simulink model "ZT_VehCtrl_18B_CAN"  (R2018b)
settings: Solver=FixedStepAuto  StartTime=0.0  StopTime=inf  FixedStep=0.005  RelTol=1e-3
InitFcn:
  | mbd_mpc_consistency_checks(bdroot(gcs));
values from neighbouring files (symbols this model uses):
  BatoverTempTh = single(80)    [VCU_INIT.m]
  BRS_PwrValid = single(5)    [VCU_INIT.m]
  BRSEnSpdTh1 = single(10)    [VCU_INIT.m]
  BRSEnSpdTh2 = single(20)    [VCU_INIT.m]
  MCUTempAlarmTh = single (60)    [VCU_INIT.m]
  mps2kmh = single(3.6)    [VCU_INIT.m]
  MtrPwrFac = single(1/9550)    [VCU_INIT.m]
  MtrTempAlarmTh = single (50)    [VCU_INIT.m]
  Padle1Signal1_Th = [PadleSignal1_min,PadleSignal1_max]    [VCU_INIT.m]
  Padle1Signal2_Th = [PadleSignal2_min,PadleSignal2_max]    [VCU_INIT.m]
  PadleSignal1_max = 3.84    [VCU_INIT.m]
  PadleSignal1_min = 0.75    [VCU_INIT.m]
  PadleSignal2_max = 1.92    [VCU_INIT.m]
  PadleSignal2_min = 0.375    [VCU_INIT.m]
  PadleValid = 0.05    [VCU_INIT.m]
  PwrLimFactor = single(0.5)    [VCU_INIT.m]
  Ratio = single(1)    [VCU_INIT.m]
  rpm2mps = single(2*pi/60 * WhlRadius/Ratio)    [VCU_INIT.m]
  SOCLowTh = single(20)    [VCU_INIT.m]
  VehPwrBackwardMax = VehPwrMax * single(0.3)    [VCU_INIT.m]
  VehPwrMax = single(MtrPwrMax * 4)    [VCU_INIT.m]
  VehTrqBackwardMax = VehTrqMax * single(0.3)    [VCU_INIT.m]
  VehTrqMax = single(MtrTrqMax * Ratio *4)    [VCU_INIT.m]
  WhlRadius = single(1)    [VCU_INIT.m]
undefined symbols (not defined in the file or in its folder): Delay_Charge, Delay_Discharge, fifo_0_vect, fifo_1_vect, LQFP, pts1_fifo_0_vect, pts1_fifo_1_vect, pts2_fifo_0_vect, pts2_fifo_1_vect, pts3_fifo_0_vect, pts3_fifo_1_vect, pts4_fifo_0_vect, pts4_fifo_1_vect
libraries: mbd_mpc574x_ec_toolbox x157, canmsglib x74, simulink x38
(part 8 of 12)

== system ZT_VehCtrl_18B_CAN/SigIn/CAN0 /BMS Statistic_Cell ExtremumIndex Infor/UNPACK ==
  ID : Inport
  data : Inport  Port=2
  length : Inport  Port=3
  timestamp : Inport  Port=4
  Action Port : ActionPort
  Bus Creator : BusCreator  Inputs=7  OutDataTypeStr=Bus: CAN_MESSAGE_BUS  NonVirtualBus=on
  Bus Creator1 : BusCreator  Inputs=2
  CAN Unpack6 : canmsglib/CAN Unpack  CANdbFile=D:\VCU\VCU_SL_ZhengZhou\ZT2\模型与接口\CAN_DBC\整车CANA_GBK.dbc  MsgList=(none)  MsgName=BMS_Statistic_Cell_ExtremumIndex  MsgIDType=Standard (11-bit identifier)  MsgIdentifier=856  MsgLength=8  SignalInfo=Statistic_CellHVMaxBatIndex$8$8$2$2$1$0$1$0$0$255$#Statistic_CellHVMaxBmsIndex$0$8$2$2$1$0$1$0$0$255$#Statistic_CellHtMaxBatIndex$40$8$2$2$1$0$1$0$0$255$#Statistic_CellHtMaxBmsIndex$32$8$2$2$1$0$1$0$0$255$#Statistic_CellLVMaxBatIndex$24$8$2$2$1$0$1$0$0$255$#Statistic_CellLVMaxBmsIndex$16$8$2$2$1$0$1$0$0$255$#Statistic_CellLtMaxBatIndex$56$8$2$2$1$0$1$0$0$255$#Statistic_CellLtMaxBmsIndex$48$8$2$2$1$0$1$0$0$255$#  NSignals=8  IDPort=off  TimestampPort=off  ErrorPort=off  RemotePort=off  LengthPort=off  StatusPort=off  StartBits=str2num('[int32(8);int32(0);int32(40);int32(32);int32(24);int32(16);int32(56);int32(48)]')  SignalSizes=str2num('[int32(8);int32(8);int32(8);int32(8);int32(8);int32(8);int32(8);int32(8)]')  ByteOrders=str2num('[int32(2);int32(2);int32(2);int32(2);int32(2);int32(2);int32(2);int32(2)]')  DataTypes=str2num('[int32(2);int32(2);int32(2);int32(2);int32(2);int32(2);int32(2);int32(2)]')  MultiplexTypes=str2num('[int32(1);int32(1);int32(1);int32(1);int32(1);int32(1);int32(1);int32(1)]')  MultiplexValues=str2num('[double(0);double(0);double(0);double(0);double(0);double(0);double(0);double(0)]')  Factors=str2num('[double(1);double(1);double(1);double(1);double(1);double(1);double(1);double(1)]')  Offsets=str2num('[double(0);double(0);double(0);double(0);double(0);double(0);double(0);double(0)]')  Minimums=str2num('[double(0);double(0);double(0);double(0);double(0);double(0);double(0);double(0)]')  Maximums=str2num('[double(255);double(255);double(255);double(255);double(255);double(255);double(255);double(255)]')  ApplyMinMax=off
      settings: SourceProductName=Simulink Real-Time  SourceProductBaseCode=XP  DataFormat=CANdb specified signals
  Constant1 : Constant  Value=0  OutDataTypeStr=uint8
  Constant4 : Constant  Value=0  OutDataTypeStr=uint8
  Constant5 : Constant  Value=0  OutDataTypeStr=uint8
  Data Type Conversion{,14..15,17} (4 alike) : DataTypeConversion  OutDataTypeStr=uint8
  Data Type Conversion18 : DataTypeConversion  OutDataTypeStr=uint32
  Data Type Conversion19 : DataTypeConversion  OutDataTypeStr=double
  Message : Outport
  wires:
  Bus Creator1/1 -> Message/1
  Data Type Conversion15/1 -> Bus Creator/3  "Remote"
  Data Type Conversion14/1 -> Bus Creator/2  "Length"
  Data Type Conversion/1 -> Bus Creator/1  "Extended"
  Bus Creator/1 -> CAN Unpack6/1  "CAN_Msg_In"
  Data Type Conversion17/1 -> Bus Creator/4  "Error"
  timestamp/1 -> Data Type Conversion19/1
  Data Type Conversion19/1 -> Bus Creator/6  "Timestamp"
  ID/1 -> Data Type Conversion18/1
  Constant5/1 -> Data Type Conversion17/1
  Constant1/1 -> Data Type Conversion/1
  Data Type Conversion18/1 -> Bus Creator/5  "ID"
  data/1 -> Bus Creator/7  "Data"
  length/1 -> Data Type Conversion14/1
  Constant4/1 -> Data Type Conversion15/1

== system ZT_VehCtrl_18B_CAN/SigIn/CAN0 /BMS Statistic_Cell Voltage Infor/UNPACK ==
  ID : Inport
  data : Inport  Port=2
  length : Inport  Port=3
  timestamp : Inport  Port=4
  Action Port : ActionPort
  Bus Creator : BusCreator  Inputs=7  OutDataTypeStr=Bus: CAN_MESSAGE_BUS  NonVirtualBus=on
  Bus Creator1 : BusCreator  Inputs=8
  CAN Unpack6 : canmsglib/CAN Unpack  CANdbFile=D:\VCU\VCU_SL_ZhengZhou\ZT2\模型与接口\CAN_DBC\整车CANA_GBK.dbc  MsgList=(none)  MsgName=BMS_Statistic_Cell_Voltage_Infor  MsgIDType=Standard (11-bit identifier)  MsgIdentifier=850  MsgLength=8  SignalInfo=Statistic_CellHVMax$8$16$2$2$1$0$1.000000e-03$0$0$10$#Statistic_CellHVMaxNum$24$16$2$2$1$0$1$0$0$1000$#Statistic_CellLVMax$40$16$2$2$1$0$1.000000e-03$0$0$10$#Statistic_CellLVMaxNum$56$16$2$2$1$0$1$0$0$1000$#  NSignals=4  IDPort=off  TimestampPort=off  ErrorPort=off  RemotePort=off  LengthPort=off  StatusPort=off  StartBits=str2num('[int32(8);int32(24);int32(40);int32(56)]')  SignalSizes=str2num('[int32(16);int32(16);int32(16);int32(16)]')  ByteOrders=str2num('[int32(2);int32(2);int32(2);int32(2)]')  DataTypes=str2num('[int32(2);int32(2);int32(2);int32(2)]')  MultiplexTypes=str2num('[int32(1);int32(1);int32(1);int32(1)]')  MultiplexValues=str2num('[double(0);double(0);double(0);double(0)]')  Factors=str2num('[double(1.000000e-03);double(1);double(1.000000e-03);double(1)]')  Offsets=str2num('[double(0);double(0);double(0);double(0)]')  Minimums=str2num('[double(0);double(0);double(0);double(0)]')  Maximums=str2num('[double(10);double(1000);double(10);double(1000)]')  ApplyMinMax=off
      settings: SourceProductName=Simulink Real-Time  SourceProductBaseCode=XP  DataFormat=CANdb specified signals
  Constant1 : Constant  Value=0  OutDataTypeStr=uint8
  Constant4 : Constant  Value=0  OutDataTypeStr=uint8
  Constant5 : Constant  Value=0  OutDataTypeStr=uint8
  Data Type Conversion{,14..15,17} (4 alike) : DataTypeConversion  OutDataTypeStr=uint8
  Data Type Conversion18 : DataTypeConversion  OutDataTypeStr=uint32
  Data Type Conversion19 : DataTypeConversion  OutDataTypeStr=double
  Message : Outport
  wires:
  Bus Creator1/1 -> Message/1
  Data Type Conversion15/1 -> Bus Creator/3  "Remote"
  Data Type Conversion14/1 -> Bus Creator/2  "Length"
  Data Type Conversion/1 -> Bus Creator/1  "Extended"
  Bus Creator/1 -> CAN Unpack6/1  "CAN_Msg_In"
  Data Type Conversion17/1 -> Bus Creator/4  "Error"
  timestamp/1 -> Data Type Conversion19/1
  Data Type Conversion19/1 -> Bus Creator/6  "Timestamp"
  ID/1 -> Data Type Conversion18/1
  Constant5/1 -> Data Type Conversion17/1
  Constant1/1 -> Data Type Conversion/1
  Data Type Conversion18/1 -> Bus Creator/5  "ID"
  data/1 -> Bus Creator/7  "Data"
  length/1 -> Data Type Conversion14/1
  Constant4/1 -> Data Type Conversion15/1

== system ZT_VehCtrl_18B_CAN/SigIn/CAN0 /BMS Statistic_HeatingTemperature/UNPACK ==
  ID : Inport
  data : Inport  Port=2
  length : Inport  Port=3
  timestamp : Inport  Port=4
  Action Port : ActionPort
  Bus Creator : BusCreator  Inputs=7  OutDataTypeStr=Bus: CAN_MESSAGE_BUS  NonVirtualBus=on
  Bus Creator1 : BusCreator  Inputs=5
  CAN Unpack6 : canmsglib/CAN Unpack  CANdbFile=D:\VCU\VCU_SL_ZhengZhou\ZT2\模型与接口\CAN_DBC\整车CANA_GBK.dbc  MsgList=(none)  MsgName=BMS_Statistic_HeatingTemperature  MsgIDType=Standard (11-bit identifier)  MsgIdentifier=852  MsgLength=8  SignalInfo=Statistic_HeatingTemperatureHTMax$0$8$2$2$1$0$1$-50$-50$125$#Statistic_HeatingTemperatureHTMaxNum$16$16$2$2$1$0$1$0$0$1000$#Statistic_HeatingTemperatureLTMax$24$8$2$2$1$0$1$-50$-50$125$#Statistic_HeatingTemperatureLTMaxNum$40$16$2$2$1$0$1$0$0$1000$#  NSignals=4  IDPort=off  TimestampPort=off  ErrorPort=off  RemotePort=off  LengthPort=off  StatusPort=off  StartBits=str2num('[int32(0);int32(16);int32(24);int32(40)]')  SignalSizes=str2num('[int32(8);int32(16);int32(8);int32(16)]')  ByteOrders=str2num('[int32(2);int32(2);int32(2);int32(2)]')  DataTypes=str2num('[int32(2);int32(2);int32(2);int32(2)]')  MultiplexTypes=str2num('[int32(1);int32(1);int32(1);int32(1)]')  MultiplexValues=str2num('[double(0);double(0);double(0);double(0)]')  Factors=str2num('[double(1);double(1);double(1);double(1)]')  Offsets=str2num('[double(-50);double(0);double(-50);double(0)]')  Minimums=str2num('[double(-50);double(0);double(-50);double(0)]')  Maximums=str2num('[double(125);double(1000);double(125);double(1000)]')  ApplyMinMax=off
      settings: SourceProductName=Simulink Real-Time  SourceProductBaseCode=XP  DataFormat=CANdb specified signals
  Constant1 : Constant  Value=0  OutDataTypeStr=uint8
  Constant4 : Constant  Value=0  OutDataTypeStr=uint8
  Constant5 : Constant  Value=0  OutDataTypeStr=uint8
  Data Type Conversion{,14..15,17} (4 alike) : DataTypeConversion  OutDataTypeStr=uint8
  Data Type Conversion18 : DataTypeConversion  OutDataTypeStr=uint32
  Data Type Conversion19 : DataTypeConversion  OutDataTypeStr=double
  Message : Outport
  wires:
  Data Type Conversion15/1 -> Bus Creator/3  "Remote"
  Data Type Conversion14/1 -> Bus Creator/2  "Length"
  Data Type Conversion/1 -> Bus Creator/1  "Extended"
  Bus Creator/1 -> CAN Unpack6/1  "CAN_Msg_In"
  Data Type Conversion17/1 -> Bus Creator/4  "Error"
  timestamp/1 -> Data Type Conversion19/1
  Data Type Conversion19/1 -> Bus Creator/6  "Timestamp"
  ID/1 -> Data Type Conversion18/1
  Constant5/1 -> Data Type Conversion17/1
  Constant1/1 -> Data Type Conversion/1
  Data Type Conversion18/1 -> Bus Creator/5  "ID"
  data/1 -> Bus Creator/7  "Data"
  length/1 -> Data Type Conversion14/1
  Constant4/1 -> Data Type Conversion15/1
  Bus Creator1/1 -> Message/1

== system ZT_VehCtrl_18B_CAN/SigIn/CAN0 /BMS Statistic_PoleTemperature/UNPACK ==
  ID : Inport
  data : Inport  Port=2
  length : Inport  Port=3
  timestamp : Inport  Port=4
  Action Port : ActionPort
  Bus Creator : BusCreator  Inputs=7  OutDataTypeStr=Bus: CAN_MESSAGE_BUS  NonVirtualBus=on
  Bus Creator1 : BusCreator  Inputs=4
  CAN Unpack6 : canmsglib/CAN Unpack  CANdbFile=D:\VCU\VCU_SL_ZhengZhou\ZT2\模型与接口\CAN_DBC\整车CANA_GBK.dbc  MsgList=(none)  MsgName=BMS_Cell_Pole_Temperature  MsgIDType=Standard (11-bit identifier)  MsgIdentifier=1012  MsgLength=8  SignalInfo=CellPoleTempearture_T1$16$8$2$2$1$0$1$-50$-50$125$#CellPoleTempearture_T2$24$8$2$2$1$0$1$-50$-50$125$#CellPoleTempearture_T3$32$8$2$2$1$0$1$-50$-50$125$#CellPoleTempearture_T4$40$8$2$2$1$0$1$-50$-50$125$#CellPoleTempearture_T5$48$8$2$2$1$0$1$-50$-50$125$#CellPoleTempearture_T6$56$8$2$2$1$0$1$-50$-50$125$#CellPoleTemperature_StartNum$8$16$2$2$1$0$1$0$0$1000$#  NSignals=7  IDPort=off  TimestampPort=off  ErrorPort=off  RemotePort=off  LengthPort=off  StatusPort=off  StartBits=str2num('[int32(16);int32(24);int32(32);int32(40);int32(48);int32(56);int32(8)]')  SignalSizes=str2num('[int32(8);int32(8);int32(8);int32(8);int32(8);int32(8);int32(16)]')  ByteOrders=str2num('[int32(2);int32(2);int32(2);int32(2);int32(2);int32(2);int32(2)]')  DataTypes=str2num('[int32(2);int32(2);int32(2);int32(2);int32(2);int32(2);int32(2)]')  MultiplexTypes=str2num('[int32(1);int32(1);int32(1);int32(1);int32(1);int32(1);int32(1)]')  MultiplexValues=str2num('[double(0);double(0);double(0);double(0);double(0);double(0);double(0)]')  Factors=str2num('[double(1);double(1);double(1);double(1);double(1);double(1);double(1)]')  Offsets=str2num('[double(-50);double(-50);double(-50);double(-50);double(-50);double(-50);double(0)]')  Minimums=str2num('[double(-50);double(-50);double(-50);double(-50);double(-50);double(-50);double(0)]')  Maximums=str2num('[double(125);double(125);double(125);double(125);double(125);double(125);double(1000)]')  ApplyMinMax=off
      settings: SourceProductName=Simulink Real-Time  SourceProductBaseCode=XP  DataFormat=CANdb specified signals
  Constant1 : Constant  Value=0  OutDataTypeStr=uint8
  Constant4 : Constant  Value=0  OutDataTypeStr=uint8
  Constant5 : Constant  Value=0  OutDataTypeStr=uint8
  Data Type Conversion{,14..15,17} (4 alike) : DataTypeConversion  OutDataTypeStr=uint8
  Data Type Conversion18 : DataTypeConversion  OutDataTypeStr=uint32
  Data Type Conversion19 : DataTypeConversion  OutDataTypeStr=double
  Message : Outport
  wires:
  Bus Creator1/1 -> Message/1
  Data Type Conversion15/1 -> Bus Creator/3  "Remote"
  Data Type Conversion14/1 -> Bus Creator/2  "Length"
  Data Type Conversion/1 -> Bus Creator/1  "Extended"
  Bus Creator/1 -> CAN Unpack6/1  "CAN_Msg_In"
  Data Type Conversion17/1 -> Bus Creator/4  "Error"
  timestamp/1 -> Data Type Conversion19/1
  Data Type Conversion19/1 -> Bus Creator/6  "Timestamp"
  ID/1 -> Data Type Conversion18/1
  Constant5/1 -> Data Type Conversion17/1
  Constant1/1 -> Data Type Conversion/1
  Data Type Conversion18/1 -> Bus Creator/5  "ID"
  data/1 -> Bus Creator/7  "Data"
  length/1 -> Data Type Conversion14/1
  Constant4/1 -> Data Type Conversion15/1

== system ZT_VehCtrl_18B_CAN/SigIn/CAN0 /BMS Statistic_Temperature of Battery/UNPACK ==
  ID : Inport
  data : Inport  Port=2
  length : Inport  Port=3
  timestamp : Inport  Port=4
  Action Port : ActionPort  ActionType=case
  Add : Sum
  Bus Creator : BusCreator  Inputs=7  OutDataTypeStr=Bus: CAN_MESSAGE_BUS  NonVirtualBus=on
  Bus Creator1 : BusCreator  Inputs=4
  CAN Unpack6 : canmsglib/CAN Unpack  CANdbFile=D:\VCU\VCU_SL_ZhengZhou\ZT2\模型与接口\CAN_DBC\整车CANA_GBK.dbc  MsgList=(none)  MsgName=BMS_Statistic_Temperature_of_Bat  MsgIDType=Standard (11-bit identifier)  MsgIdentifier=851  MsgLength=8  SignalInfo=Statistic_TemperatureHTMax$0$8$2$2$1$0$1$-50$-50$125$#Statistic_TemperatureHTMaxNum$16$16$2$2$1$0$1$0$1$1000$#Statistic_TemperatureLTMax$24$8$2$2$1$0$1$-50$-50$125$#Statistic_TemperatureLTMaxNum$40$16$2$2$1$0$1$0$1$1000$#  NSignals=4  IDPort=off  TimestampPort=off  ErrorPort=off  RemotePort=off  LengthPort=off  StatusPort=off  StartBits=str2num('[int32(0);int32(16);int32(24);int32(40)]')  SignalSizes=str2num('[int32(8);int32(16);int32(8);int32(16)]')  ByteOrders=str2num('[int32(2);int32(2);int32(2);int32(2)]')  DataTypes=str2num('[int32(2);int32(2);int32(2);int32(2)]')  MultiplexTypes=str2num('[int32(1);int32(1);int32(1);int32(1)]')  MultiplexValues=str2num('[double(0);double(0);double(0);double(0)]')  Factors=str2num('[double(1);double(1);double(1);double(1)]')  Offsets=str2num('[double(-50);double(0);double(-50);double(0)]')  Minimums=str2num('[double(-50);double(1);double(-50);double(1)]')  Maximums=str2num('[double(125);double(1000);double(125);double(1000)]')  ApplyMinMax=off
      settings: SourceProductName=Simulink Real-Time  SourceProductBaseCode=XP  DataFormat=CANdb specified signals
  Constant : Constant  OutDataTypeStr=uint8
  Constant1 : Constant  Value=0  OutDataTypeStr=uint8
  Constant4 : Constant  Value=0  OutDataTypeStr=uint8
  Constant5 : Constant  Value=0  OutDataTypeStr=uint8
  Data Store Read : DataStoreRead  DataStoreName=Cnt_BMS5
  Data Store Write : DataStoreWrite  DataStoreName=Cnt_BMS5
  Data Type Conversion{,14..15,17} (4 alike) : DataTypeConversion  OutDataTypeStr=uint8
  Data Type Conversion{1..4} (4 alike) : DataTypeConversion  OutDataTypeStr=single
  Data Type Conversion18 : DataTypeConversion  OutDataTypeStr=uint32
  Data Type Conversion19 : DataTypeConversion  OutDataTypeStr=double
  Message : Outport
  wires:
  Bus Creator1/1 -> Message/1
  Data Type Conversion15/1 -> Bus Creator/3  "Remote"
  Data Type Conversion14/1 -> Bus Creator/2  "Length"
  Data Type Conversion/1 -> Bus Creator/1  "Extended"
  Bus Creator/1 -> CAN Unpack6/1  "CAN_Msg_In"
  Data Type Conversion17/1 -> Bus Creator/4  "Error"
  timestamp/1 -> Data Type Conversion19/1
  Data Type Conversion19/1 -> Bus Creator/6  "Timestamp"
  ID/1 -> Data Type Conversion18/1
  Constant5/1 -> Data Type Conversion17/1
  Constant1/1 -> Data Type Conversion/1
  Data Type Conversion18/1 -> Bus Creator/5  "ID"
  data/1 -> Bus Creator/7  "Data"
  length/1 -> Data Type Conversion14/1
  Constant4/1 -> Data Type Conversion15/1
  CAN Unpack6/1 -> Data Type Conversion1/1
  CAN Unpack6/2 -> Data Type Conversion2/1
  CAN Unpack6/3 -> Data Type Conversion3/1
  CAN Unpack6/4 -> Data Type Conversion4/1
  Data Type Conversion1/1 -> Bus Creator1/1  "Statistic_TemperatureHTMax"
  Data Type Conversion2/1 -> Bus Creator1/2  "Statistic_TemperatureHTMaxNum"
  Data Type Conversion3/1 -> Bus Creator1/3  "Statistic_TemperatureLTMax"
  Data Type Conversion4/1 -> Bus Creator1/4  "Statistic_TemperatureLTMaxNum"
  Data Store Read/1 -> Add/1
  Constant/1 -> Add/2
  Add/1 -> Data Store Write/1

== system ZT_VehCtrl_18B_CAN/SigIn/CAN0 /BMS _SystemTime /UNPACK ==
  ID : Inport
  data : Inport  Port=2
  length : Inport  Port=3
  timestamp : Inport  Port=4
  Action Port : ActionPort
  Bus Creator : BusCreator  Inputs=7  OutDataTypeStr=Bus: CAN_MESSAGE_BUS  NonVirtualBus=on
  Bus Creator1 : BusCreator  Inputs=2
  CAN Unpack6 : canmsglib/CAN Unpack  CANdbFile=D:\VCU\VCU_SL_ZhengZhou\ZT2\模型与接口\CAN_DBC\整车CANA_GBK.dbc  MsgList=(none)  MsgName=BMS_SystemTime  MsgIDType=Standard (11-bit identifier)  MsgIdentifier=514  MsgLength=8  SignalInfo=System_Day$24$8$2$2$1$0$1$0$0$31$#System_Hour$32$8$2$2$1$0$1$0$0$23$#System_Minute$40$8$2$2$1$0$1$0$0$59$#System_Month$16$8$2$2$1$0$1$0$0$12$#System_Seconds$48$8$2$2$1$0$1$0$0$59$#System_Year$8$16$2$2$1$0$1$0$0$65535$#  NSignals=6  IDPort=off  TimestampPort=off  ErrorPort=off  RemotePort=off  LengthPort=off  StatusPort=off  StartBits=str2num('[int32(24);int32(32);int32(40);int32(16);int32(48);int32(8)]')  SignalSizes=str2num('[int32(8);int32(8);int32(8);int32(8);int32(8);int32(16)]')  ByteOrders=str2num('[int32(2);int32(2);int32(2);int32(2);int32(2);int32(2)]')  DataTypes=str2num('[int32(2);int32(2);int32(2);int32(2);int32(2);int32(2)]')  MultiplexTypes=str2num('[int32(1);int32(1);int32(1);int32(1);int32(1);int32(1)]')  MultiplexValues=str2num('[double(0);double(0);double(0);double(0);double(0);double(0)]')  Factors=str2num('[double(1);double(1);double(1);double(1);double(1);double(1)]')  Offsets=str2num('[double(0);double(0);double(0);double(0);double(0);double(0)]')  Minimums=str2num('[double(0);double(0);double(0);double(0);double(0);double(0)]')  Maximums=str2num('[double(31);double(23);double(59);double(12);double(59);double(65535)]')  ApplyMinMax=off
      settings: SourceProductName=Simulink Real-Time  SourceProductBaseCode=XP  DataFormat=CANdb specified signals
  Constant1 : Constant  Value=0  OutDataTypeStr=uint8
  Constant4 : Constant  Value=0  OutDataTypeStr=uint8
  Constant5 : Constant  Value=0  OutDataTypeStr=uint8
  Data Type Conversion{,14..15,17} (4 alike) : DataTypeConversion  OutDataTypeStr=uint8
  Data Type Conversion18 : DataTypeConversion  OutDataTypeStr=uint32
  Data Type Conversion19 : DataTypeConversion  OutDataTypeStr=double
  Message : Outport
  wires:
  Constant4/1 -> Data Type Conversion15/1
  length/1 -> Data Type Conversion14/1
  data/1 -> Bus Creator/7  "Data"
  Data Type Conversion18/1 -> Bus Creator/5  "ID"
  Constant1/1 -> Data Type Conversion/1
  Constant5/1 -> Data Type Conversion17/1
  ID/1 -> Data Type Conversion18/1
  Data Type Conversion19/1 -> Bus Creator/6  "Timestamp"
  timestamp/1 -> Data Type Conversion19/1
  Data Type Conversion17/1 -> Bus Creator/4  "Error"
  Bus Creator/1 -> CAN Unpack6/1  "CAN_Msg_In"
  Data Type Conversion/1 -> Bus Creator/1  "Extended"
  Data Type Conversion14/1 -> Bus Creator/2  "Length"
  Data Type Conversion15/1 -> Bus Creator/3  "Remote"
  Bus Creator1/1 -> Message/1

== system ZT_VehCtrl_18B_CAN/SigIn/CAN0 /BMS other Information1/UNPACK ==
  ID : Inport
  data : Inport  Port=2
  length : Inport  Port=3
  timestamp : Inport  Port=4
  Action Port : ActionPort
  Bus Creator : BusCreator  Inputs=7  OutDataTypeStr=Bus: CAN_MESSAGE_BUS  NonVirtualBus=on
  Bus Creator1 : BusCreator  Inputs=2
  CAN Unpack6 : canmsglib/CAN Unpack  CANdbFile=D:\VCU\VCU_SL_ZhengZhou\ZT2\模型与接口\CAN_DBC\整车CANA_GBK.dbc  MsgList=(none)  MsgName=BMS_other_Information1  MsgIDType=Standard (11-bit identifier)  MsgIdentifier=1014  MsgLength=8  SignalInfo=Statistic_AverageTemperature$16$8$2$2$1$0$1$-50$-50$125$#Statistic_AverageVoltage$8$16$2$2$1$0$1.000000e-03$0$0$10$#Statistic_ChargeTimes$56$16$2$2$1$0$1$0$-Inf$Inf$#Statistic_DeltaTemperature$40$8$2$2$1$0$1$-50$-50$125$#Statistic_DeltaVoltage$32$16$2$2$1$0$1.000000e-03$0$0$10$#  NSignals=5  IDPort=off  TimestampPort=off  ErrorPort=off  RemotePort=off  LengthPort=off  StatusPort=off  StartBits=str2num('[int32(16);int32(8);int32(56);int32(40);int32(32)]')  SignalSizes=str2num('[int32(8);int32(16);int32(16);int32(8);int32(16)]')  ByteOrders=str2num('[int32(2);int32(2);int32(2);int32(2);int32(2)]')  DataTypes=str2num('[int32(2);int32(2);int32(2);int32(2);int32(2)]')  MultiplexTypes=str2num('[int32(1);int32(1);int32(1);int32(1);int32(1)]')  MultiplexValues=str2num('[double(0);double(0);double(0);double(0);double(0)]')  Factors=str2num('[double(1);double(1.000000e-03);double(1);double(1);double(1.000000e-03)]')  Offsets=str2num('[double(-50);double(0);double(0);double(-50);double(0)]')  Minimums=str2num('[double(-50);double(0);double(-Inf);double(-50);double(0)]')  Maximums=str2num('[double(125);double(10);double(Inf);double(125);double(10)]')  ApplyMinMax=off
      settings: SourceProductName=Simulink Real-Time  SourceProductBaseCode=XP  DataFormat=CANdb specified signals
  Constant1 : Constant  Value=0  OutDataTypeStr=uint8
  Constant4 : Constant  Value=0  OutDataTypeStr=uint8
  Constant5 : Constant  Value=0  OutDataTypeStr=uint8
  Data Type Conversion{,14..15,17} (4 alike) : DataTypeConversion  OutDataTypeStr=uint8
  Data Type Conversion18 : DataTypeConversion  OutDataTypeStr=uint32
  Data Type Conversion19 : DataTypeConversion  OutDataTypeStr=double
  Message : Outport
  wires:
  Bus Creator1/1 -> Message/1
  Data Type Conversion15/1 -> Bus Creator/3  "Remote"
  Data Type Conversion14/1 -> Bus Creator/2  "Length"
  Data Type Conversion/1 -> Bus Creator/1  "Extended"
  Bus Creator/1 -> CAN Unpack6/1  "CAN_Msg_In"
  Data Type Conversion17/1 -> Bus Creator/4  "Error"
  timestamp/1 -> Data Type Conversion19/1
  Data Type Conversion19/1 -> Bus Creator/6  "Timestamp"
  ID/1 -> Data Type Conversion18/1
  Constant5/1 -> Data Type Conversion17/1
  Constant1/1 -> Data Type Conversion/1
  Data Type Conversion18/1 -> Bus Creator/5  "ID"
  data/1 -> Bus Creator/7  "Data"
  length/1 -> Data Type Conversion14/1
  Constant4/1 -> Data Type Conversion15/1

== system ZT_VehCtrl_18B_CAN/SigIn/CAN0 /BMS other Information2 /UNPACK ==
  ID : Inport
  data : Inport  Port=2
  length : Inport  Port=3
  timestamp : Inport  Port=4
  Action Port : ActionPort
  Bus Creator : BusCreator  Inputs=7  OutDataTypeStr=Bus: CAN_MESSAGE_BUS  NonVirtualBus=on
  Bus Creator1 : BusCreator  Inputs=2
  CAN Unpack6 : canmsglib/CAN Unpack  CANdbFile=D:\VCU\VCU_SL_ZhengZhou\ZT2\模型与接口\CAN_DBC\整车CANA_GBK.dbc  MsgList=(none)  MsgName=BMS_other_Information2  MsgIDType=Standard (11-bit identifier)  MsgIdentifier=1023  MsgLength=8  SignalInfo=CellTemp_Number$24$16$2$2$1$0$1$0$0$255$#Cell_Number$8$16$2$2$1$0$1$0$0$1000$#HeatTemp_Numer$56$16$2$2$1$0$1$1$0$255$#PoleTemp_Number$40$16$2$2$1$0$1$0$0$255$#  NSignals=4  IDPort=off  TimestampPort=off  ErrorPort=off  RemotePort=off  LengthPort=off  StatusPort=off  StartBits=str2num('[int32(24);int32(8);int32(56);int32(40)]')  SignalSizes=str2num('[int32(16);int32(16);int32(16);int32(16)]')  ByteOrders=str2num('[int32(2);int32(2);int32(2);int32(2)]')  DataTypes=str2num('[int32(2);int32(2);int32(2);int32(2)]')  MultiplexTypes=str2num('[int32(1);int32(1);int32(1);int32(1)]')  MultiplexValues=str2num('[double(0);double(0);double(0);double(0)]')  Factors=str2num('[double(1);double(1);double(1);double(1)]')  Offsets=str2num('[double(0);double(0);double(1);double(0)]')  Minimums=str2num('[double(0);double(0);double(0);double(0)]')  Maximums=str2num('[double(255);double(1000);double(255);double(255)]')  ApplyMinMax=off
      settings: SourceProductName=Simulink Real-Time  SourceProductBaseCode=XP  DataFormat=CANdb specified signals
  Constant1 : Constant  Value=0  OutDataTypeStr=uint8
  Constant4 : Constant  Value=0  OutDataTypeStr=uint8
  Constant5 : Constant  Value=0  OutDataTypeStr=uint8
  Data Type Conversion{,14..15,17} (4 alike) : DataTypeConversion  OutDataTypeStr=uint8
  Data Type Conversion18 : DataTypeConversion  OutDataTypeStr=uint32
  Data Type Conversion19 : DataTypeConversion  OutDataTypeStr=double
  Message : Outport
  wires:
  Constant4/1 -> Data Type Conversion15/1
  length/1 -> Data Type Conversion14/1
  data/1 -> Bus Creator/7  "Data"
  Data Type Conversion18/1 -> Bus Creator/5  "ID"
  Constant1/1 -> Data Type Conversion/1
  Constant5/1 -> Data Type Conversion17/1
  ID/1 -> Data Type Conversion18/1
  Data Type Conversion19/1 -> Bus Creator/6  "Timestamp"
  timestamp/1 -> Data Type Conversion19/1
  Data Type Conversion17/1 -> Bus Creator/4  "Error"
  Bus Creator/1 -> CAN Unpack6/1  "CAN_Msg_In"
  Data Type Conversion/1 -> Bus Creator/1  "Extended"
  Data Type Conversion14/1 -> Bus Creator/2  "Length"
  Data Type Conversion15/1 -> Bus Creator/3  "Remote"
  Bus Creator1/1 -> Message/1

== system ZT_VehCtrl_18B_CAN/SigIn/CAN0 /BMS other Information3/UNPACK ==
  ID : Inport
  data : Inport  Port=2
  length : Inport  Port=3
  timestamp : Inport  Port=4
  Action Port : ActionPort  ActionType=case
  Add : Sum
  Bus Creator : BusCreator  Inputs=7  OutDataTypeStr=Bus: CAN_MESSAGE_BUS  NonVirtualBus=on
  Bus Creator1 : BusCreator  Inputs=4
  CAN Unpack6 : canmsglib/CAN Unpack  CANdbFile=D:\VCU\VCU_SL_ZhengZhou\ZT2\Module\CAN_DBC\所有CAN信号\整车CANA_GBK.dbc  MsgList=(none)  MsgName=BMS_other_Information3  MsgIDType=Standard (11-bit identifier)  MsgIdentifier=517  MsgLength=8  SignalInfo=Charge_Time$40$16$2$2$1$0$1$0$0$6.553500e+03$#Pack_LeftCap$24$16$2$2$1$0$1.000000e-01$0$-Inf$Inf$#Pack_TotalCap$8$16$2$2$1$0$1.000000e-01$0$-Inf$Inf$#SOH$56$16$2$2$1$0$1.000000e-01$0$0$100$#  NSignals=4  IDPort=off  TimestampPort=off  ErrorPort=off  RemotePort=off  LengthPort=off  StatusPort=off  StartBits=str2num('[int32(40);int32(24);int32(8);int32(56)]')  SignalSizes=str2num('[int32(16);int32(16);int32(16);int32(16)]')  ByteOrders=str2num('[int32(2);int32(2);int32(2);int32(2)]')  DataTypes=str2num('[int32(2);int32(2);int32(2);int32(2)]')  MultiplexTypes=str2num('[int32(1);int32(1);int32(1);int32(1)]')  MultiplexValues=str2num('[double(0);double(0);double(0);double(0)]')  Factors=str2num('[double(1);double(1.000000e-01);double(1.000000e-01);double(1.000000e-01)]')  Offsets=str2num('[double(0);double(0);double(0);double(0)]')  Minimums=str2num('[double(0);double(-Inf);double(-Inf);double(0)]')  Maximums=str2num('[double(6.553500e+03);double(Inf);double(Inf);double(100)]')  ApplyMinMax=off
      settings: SourceProductName=Simulink Real-Time  SourceProductBaseCode=XP  DataFormat=CANdb specified signals
  Constant : Constant  OutDataTypeStr=uint8
  Constant1 : Constant  Value=0  OutDataTypeStr=uint8
  Constant4 : Constant  Value=0  OutDataTypeStr=uint8
  Constant5 : Constant  Value=0  OutDataTypeStr=uint8
  Data Store Read : DataStoreRead  DataStoreName=Cnt_BMS6
  Data Store Write : DataStoreWrite  DataStoreName=Cnt_BMS6
  Data Type Conversion{,14..15,17} (4 alike) : DataTypeConversion  OutDataTypeStr=uint8
  Data Type Conversion{1..4} (4 alike) : DataTypeConversion  OutDataTypeStr=single
  Data Type Conversion18 : DataTypeConversion  OutDataTypeStr=uint32
  Data Type Conversion19 : DataTypeConversion  OutDataTypeStr=double
  Message : Outport
  wires:
  Bus Creator1/1 -> Message/1
  Data Type Conversion15/1 -> Bus Creator/3  "Remote"
  Data Type Conversion14/1 -> Bus Creator/2  "Length"
  Data Type Conversion/1 -> Bus Creator/1  "Extended"
  Bus Creator/1 -> CAN Unpack6/1  "CAN_Msg_In"
  Data Type Conversion17/1 -> Bus Creator/4  "Error"
  timestamp/1 -> Data Type Conversion19/1
  Data Type Conversion19/1 -> Bus Creator/6  "Timestamp"
  ID/1 -> Data Type Conversion18/1
  Constant5/1 -> Data Type Conversion17/1
  Constant1/1 -> Data Type Conversion/1
  Data Type Conversion18/1 -> Bus Creator/5  "ID"
  data/1 -> Bus Creator/7  "Data"
  length/1 -> Data Type Conversion14/1
  Constant4/1 -> Data Type Conversion15/1
  CAN Unpack6/1 -> Data Type Conversion4/1
  CAN Unpack6/2 -> Data Type Conversion1/1
  CAN Unpack6/3 -> Data Type Conversion2/1
  CAN Unpack6/4 -> Data Type Conversion3/1
  Data Type Conversion3/1 -> Bus Creator1/4  "SOH"
  Data Type Conversion2/1 -> Bus Creator1/3  "Pack_TotalCap"
  Data Type Conversion1/1 -> Bus Creator1/2  "Pack_LeftCap"
  Data Type Conversion4/1 -> Bus Creator1/1  "Charge_Time"
  Data Store Read/1 -> Add/1
  Constant/1 -> Add/2
  Add/1 -> Data Store Write/1

== system ZT_VehCtrl_18B_CAN/SigIn/CAN0 /BMSWarning_Status/UNPACK ==
  ID : Inport
  data : Inport  Port=2
  length : Inport  Port=3
  timestamp : Inport  Port=4
  Action Port : ActionPort  ActionType=case
  Add : Sum
  Bus Creator : BusCreator  Inputs=7  OutDataTypeStr=Bus: CAN_MESSAGE_BUS  NonVirtualBus=on
  Bus Creator1 : BusCreator  Inputs=2
  CAN Unpack6 : canmsglib/CAN Unpack  CANdbFile=D:\VCU\VCU_SL_ZhengZhou\ZT2\模型与接口\CAN_DBC\整车CANA_GBK.dbc  MsgList=(none)  MsgName=BMSWarning_Status  MsgIDType=Standard (11-bit identifier)  MsgIdentifier=501  MsgLength=8  SignalInfo=Alarm_Code$0$8$2$2$1$0$1$0$0$254$#Alarm_Level$8$8$2$2$1$0$1$0$0$255$#  NSignals=2  IDPort=off  TimestampPort=off  ErrorPort=off  RemotePort=off  LengthPort=off  StatusPort=off  StartBits=str2num('[int32(0);int32(8)]')  SignalSizes=str2num('[int32(8);int32(8)]')  ByteOrders=str2num('[int32(2);int32(2)]')  DataTypes=str2num('[int32(2);int32(2)]')  MultiplexTypes=str2num('[int32(1);int32(1)]')  MultiplexValues=str2num('[double(0);double(0)]')  Factors=str2num('[double(1);double(1)]')  Offsets=str2num('[double(0);double(0)]')  Minimums=str2num('[double(0);double(0)]')  Maximums=str2num('[double(254);double(255)]')  ApplyMinMax=off
      settings: SourceProductName=Simulink Real-Time  SourceProductBaseCode=XP  DataFormat=CANdb specified signals
  Constant : Constant  OutDataTypeStr=uint8
  Constant1 : Constant  Value=0  OutDataTypeStr=uint8
  Constant4 : Constant  Value=0  OutDataTypeStr=uint8
  Constant5 : Constant  Value=0  OutDataTypeStr=uint8
  Data Store Read : DataStoreRead  DataStoreName=Cnt_BMS3
  Data Store Write : DataStoreWrite  DataStoreName=Cnt_BMS3
  Data Type Conversion{,14..15,17} (4 alike) : DataTypeConversion  OutDataTypeStr=uint8
  Data Type Conversion1 : DataTypeConversion  OutDataTypeStr=single
  Data Type Conversion18 : DataTypeConversion  OutDataTypeStr=uint32
  Data Type Conversion19 : DataTypeConversion  OutDataTypeStr=double
  Data Type Conversion2 : DataTypeConversion  OutDataTypeStr=single
  Message : Outport
  wires:
  Bus Creator1/1 -> Message/1
  Data Type Conversion15/1 -> Bus Creator/3  "Remote"
  Data Type Conversion14/1 -> Bus Creator/2  "Length"
  Data Type Conversion/1 -> Bus Creator/1  "Extended"
  Bus Creator/1 -> CAN Unpack6/1  "CAN_Msg_In"
  Data Type Conversion17/1 -> Bus Creator/4  "Error"
  timestamp/1 -> Data Type Conversion19/1
  Data Type Conversion19/1 -> Bus Creator/6  "Timestamp"
  ID/1 -> Data Type Conversion18/1
  Constant5/1 -> Data Type Conversion17/1
  Constant1/1 -> Data Type Conversion/1
  Data Type Conversion18/1 -> Bus Creator/5  "ID"
  data/1 -> Bus Creator/7  "Data"
  length/1 -> Data Type Conversion14/1
  Constant4/1 -> Data Type Conversion15/1
  CAN Unpack6/2 -> Data Type Conversion2/1
  CAN Unpack6/1 -> Data Type Conversion1/1
  Data Type Conversion1/1 -> Bus Creator1/1  "Alarm_Code"
  Data Type Conversion2/1 -> Bus Creator1/2  "Alarm_Level"
  Data Store Read/1 -> Add/1
  Add/1 -> Data Store Write/1
  Constant/1 -> Add/2

== system ZT_VehCtrl_18B_CAN/SigIn/CAN0 /BMS_Information1/UNPACK ==
  ID : Inport
  data : Inport  Port=2
  length : Inport  Port=3
  timestamp : Inport  Port=4
  Action Port : ActionPort  ActionType=case
  Add : Sum
  Bus Creator : BusCreator  Inputs=7  OutDataTypeStr=Bus: CAN_MESSAGE_BUS  NonVirtualBus=on
  Bus Creator1 : BusCreator  Inputs=4
  CAN Unpack6 : canmsglib/CAN Unpack  CANdbFile=D:\VCU\VCU_SL_ZhengZhou\ZT2\模型与接口\CAN_DBC\整车CANA_GBK.dbc  MsgList=(none)  MsgName=BMS_Information_1  MsgIDType=Standard (11-bit identifier)  MsgIdentifier=481  MsgLength=8  SignalInfo=Cur_Bat$24$16$2$2$1$0$1.000000e-01$-1000$-1000$1000$#Display_SOC$56$16$2$2$1$0$1.000000e-01$0$0$100$#SOC$40$16$2$2$1$0$1.000000e-01$0$0$100$#Vol_Bat$8$16$2$2$1$0$1.000000e-01$0$0$800$#  NSignals=4  IDPort=off  TimestampPort=off  ErrorPort=off  RemotePort=off  LengthPort=off  StatusPort=off  StartBits=str2num('[int32(24);int32(56);int32(40);int32(8)]')  SignalSizes=str2num('[int32(16);int32(16);int32(16);int32(16)]')  ByteOrders=str2num('[int32(2);int32(2);int32(2);int32(2)]')  DataTypes=str2num('[int32(2);int32(2);int32(2);int32(2)]')  MultiplexTypes=str2num('[int32(1);int32(1);int32(1);int32(1)]')  MultiplexValues=str2num('[double(0);double(0);double(0);double(0)]')  Factors=str2num('[double(1.000000e-01);double(1.000000e-01);double(1.000000e-01);double(1.000000e-01)]')  Offsets=str2num('[double(-1000);double(0);double(0);double(0)]')  Minimums=str2num('[double(-1000);double(0);double(0);double(0)]')  Maximums=str2num('[double(1000);double(100);double(100);double(800)]')  ApplyMinMax=off
      settings: SourceProductName=Simulink Real-Time  SourceProductBaseCode=XP  DataFormat=CANdb specified signals
  Constant : Constant  OutDataTypeStr=uint8
  Constant1 : Constant  Value=0  OutDataTypeStr=uint8
  Constant4 : Constant  Value=0  OutDataTypeStr=uint8
  Constant5 : Constant  Value=0  OutDataTypeStr=uint8
  Data Store Read : DataStoreRead  DataStoreName=Cnt_BMS1
  Data Store Write : DataStoreWrite  DataStoreName=Cnt_BMS1
  Data Type Conversion{,14..15,17} (4 alike) : DataTypeConversion  OutDataTypeStr=uint8
  Data Type Conversion{1..4} (4 alike) : DataTypeConversion  OutDataTypeStr=single
  Data Type Conversion18 : DataTypeConversion  OutDataTypeStr=uint32
  Data Type Conversion19 : DataTypeConversion  OutDataTypeStr=double
  Message : Outport
  wires:
  Bus Creator1/1 -> Message/1
  Data Type Conversion15/1 -> Bus Creator/3  "Remote"
  Data Type Conversion14/1 -> Bus Creator/2  "Length"
  Data Type Conversion/1 -> Bus Creator/1  "Extended"
  Bus Creator/1 -> CAN Unpack6/1  "CAN_Msg_In"
  Data Type Conversion17/1 -> Bus Creator/4  "Error"
  timestamp/1 -> Data Type Conversion19/1
  Data Type Conversion19/1 -> Bus Creator/6  "Timestamp"
  ID/1 -> Data Type Conversion18/1
  Constant5/1 -> Data Type Conversion17/1
  Constant1/1 -> Data Type Conversion/1
  Data Type Conversion18/1 -> Bus Creator/5  "ID"
  data/1 -> Bus Creator/7  "Data"
  length/1 -> Data Type Conversion14/1
  Constant4/1 -> Data Type Conversion15/1
  CAN Unpack6/1 -> Data Type Conversion1/1
  CAN Unpack6/2 -> Data Type Conversion2/1
  CAN Unpack6/3 -> Data Type Conversion3/1
  CAN Unpack6/4 -> Data Type Conversion4/1
  Data Type Conversion1/1 -> Bus Creator1/1  "Cur_Bat"
  Data Type Conversion2/1 -> Bus Creator1/2  "Display_SOC"
  Data Type Conversion3/1 -> Bus Creator1/3  "SOC"
  Data Type Conversion4/1 -> Bus Creator1/4  "Vol_Bat"
  Add/1 -> Data Store Write/1
  Constant/1 -> Add/2
  Data Store Read/1 -> Add/1

== system ZT_VehCtrl_18B_CAN/SigIn/CAN0 /BMS_Information2/UNPACK ==
  ID : Inport
  data : Inport  Port=2
  length : Inport  Port=3
  timestamp : Inport  Port=4
  Action Port : ActionPort  ActionType=case
  Add : Sum
  Bus Creator : BusCreator  Inputs=7  OutDataTypeStr=Bus: CAN_MESSAGE_BUS  NonVirtualBus=on
  Bus Creator1 : BusCreator  Inputs=13
  CAN Unpack6 : canmsglib/CAN Unpack  CANdbFile=D:\VCU\VCU_SL_ZhengZhou\ZT2\模型与接口\CAN_DBC\整车CANA_GBK.dbc  MsgList=(none)  MsgName=BMS_Information_2  MsgIDType=Standard (11-bit identifier)  MsgIdentifier=484  MsgLength=8  SignalInfo=BMS_AlarmLevel$48$8$2$2$1$0$1$0$0$15$#BMS_BalanceStatus$12$1$2$2$1$0$1$0$0$1$#BMS_ChargeMode$4$2$2$2$1$0$1$0$0$3$#BMS_ChargeStatus$6$2$2$2$1$0$1$0$0$3$#BMS_HeatingStatus$13$1$2$2$1$0$1$0$0$1$#BMS_PrechargeStatus$8$2$2$2$1$0$1$0$0$3$#BMS_ReadySt$56$2$2$2$1$0$1$0$0$3$#BMS_RefrigerationStatus$14$1$2$2$1$0$1$0$0$1$#BMS_SelfCheckStatus$10$2$2$2$1$0$1$0$0$3$#BmsMode$58$1$2$2$1$0$1$0$0$1$#HighVoltLoopLockStatus$15$1$2$2$1$0$1$0$0$1$#NegativeInsulationResistance$40$16$2$2$1$0$1$0$0$60$#PositiveInsulationResistance$24$16$2$2$1$0$1$0$0$60$#  NSignals=13  IDPort=off  TimestampPort=off  ErrorPort=off  RemotePort=off  LengthPort=off  StatusPort=off  StartBits=str2num('[int32(48);int32(12);int32(4);int32(6);int32(13);int32(8);int32(56);int32(14);int32(10);int32(58);int32(15);int32(40);int32(24)]')  SignalSizes=str2num('[int32(8);int32(1);int32(2);int32(2);int32(1);int32(2);int32(2);int32(1);int32(2);int32(1);int32(1);int32(16);int32(16)]')  ByteOrders=str2num('[int32(2);int32(2);int32(2);int32(2);int32(2);int32(2);int32(2);int32(2);int32(2);int32(2);int32(2);int32(2);int32(2)]')  DataTypes=str2num('[int32(2);int32(2);int32(2);int32(2);int32(2);int32(2);int32(2);int32(2);int32(2);int32(2);int32(2);int32(2);int32(2)]')  MultiplexTypes=str2num('[int32(1);int32(1);int32(1);int32(1);int32(1);int32(1);int32(1);int32(1);int32(1);int32(1);int32(1);int32(1);int32(1)]')  MultiplexValues=str2num('[double(0);double(0);double(0);double(0);double(0);double(0);double(0);double(0);double(0);double(0);double(0);double(0);double(0)]')  Factors=str2num('[double(1);double(1);double(1);double(1);double(1);double(1);double(1);double(1);double(1);double(1);double(1);double(1);double(1)]')  Offsets=str2num('[double(0);double(0);double(0);double(0);double(0);double(0);double(0);double(0);double(0);double(0);double(0);double(0);double(0)]')  Minimums=str2num('[double(0);double(0);double(0);double(0);double(0);double(0);double(0);double(0);double(0);double(0);double(0);double(0);double(0)]')  Maximums=str2num('[double(15);double(1);double(3);double(3);double(1);double(3);double(3);double(1);double(3);double(1);double(1);double(60);double(60)]')  ApplyMinMax=off
      settings: SourceProductName=Simulink Real-Time  SourceProductBaseCode=XP  DataFormat=CANdb specified signals
  Constant : Constant  OutDataTypeStr=uint8
  Constant1 : Constant  Value=0  OutDataTypeStr=uint8
  Constant4 : Constant  Value=0  OutDataTypeStr=uint8
  Constant5 : Constant  Value=0  OutDataTypeStr=uint8
  Data Store Read : DataStoreRead  DataStoreName=Cnt_BMS2
  Data Store Write : DataStoreWrite  DataStoreName=Cnt_BMS2
  Data Type Conversion{,14..15,17} (4 alike) : DataTypeConversion  OutDataTypeStr=uint8
  Data Type Conversion{1,3..4,6..7,9,12..13} (8 alike) : DataTypeConversion  OutDataTypeStr=single
  Data Type Conversion{2,5,8,10..11} (5 alike) : DataTypeConversion  OutDataTypeStr=boolean
  Data Type Conversion18 : DataTypeConversion  OutDataTypeStr=uint32
  Data Type Conversion19 : DataTypeConversion  OutDataTypeStr=double
  Message : Outport
  wires:
  Constant4/1 -> Data Type Conversion15/1
  length/1 -> Data Type Conversion14/1
  data/1 -> Bus Creator/7  "Data"
  Data Type Conversion18/1 -> Bus Creator/5  "ID"
  Constant1/1 -> Data Type Conversion/1
  Constant5/1 -> Data Type Conversion17/1
  ID/1 -> Data Type Conversion18/1
  Data Type Conversion19/1 -> Bus Creator/6  "Timestamp"
  timestamp/1 -> Data Type Conversion19/1
  Data Type Conversion17/1 -> Bus Creator/4  "Error"
  Bus Creator/1 -> CAN Unpack6/1  "CAN_Msg_In"
  Data Type Conversion/1 -> Bus Creator/1  "Extended"
  Data Type Conversion14/1 -> Bus Creator/2  "Length"
  Data Type Conversion15/1 -> Bus Creator/3  "Remote"
  Bus Creator1/1 -> Message/1
  CAN Unpack6/1 -> Data Type Conversion1/1
  CAN Unpack6/2 -> Data Type Conversion2/1
  CAN Unpack6/3 -> Data Type Conversion3/1
  CAN Unpack6/4 -> Data Type Conversion4/1
  CAN Unpack6/5 -> Data Type Conversion5/1
  CAN Unpack6/6 -> Data Type Conversion6/1
  CAN Unpack6/7 -> Data Type Conversion7/1
  CAN Unpack6/8 -> Data Type Conversion8/1
  CAN Unpack6/9 -> Data Type Conversion9/1
  CAN Unpack6/10 -> Data Type Conversion10/1
  CAN Unpack6/11 -> Data Type Conversion11/1
  CAN Unpack6/12 -> Data Type Conversion12/1
  CAN Unpack6/13 -> Data Type Conversion13/1
  Data Type Conversion1/1 -> Bus Creator1/1  "BMS_AlarmLevel"
  Data Type Conversion2/1 -> Bus Creator1/2  "BMS_BalanceStatus"
  Data Type Conversion3/1 -> Bus Creator1/3  "BMS_ChargeMode"
  Data Type Conversion4/1 -> Bus Creator1/4  "BMS_ChargeStatus"
  Data Type Conversion5/1 -> Bus Creator1/5  "BMS_HeatingStatus"
  Data Type Conversion6/1 -> Bus Creator1/6  "BMS_PrechargeStatus"
  Data Type Conversion7/1 -> Bus Creator1/7  "BMS_ReadySt"
  Data Type Conversion8/1 -> Bus Creator1/8  "BMS_RefrigerationStatus"
  Data Type Conversion9/1 -> Bus Creator1/9  "BMS_SelfCheckStatus"
  Data Type Conversion10/1 -> Bus Creator1/10  "BmsMode"
  Data Type Conversion11/1 -> Bus Creator1/11  "HighVoltLoopLockStatus"
  Data Type Conversion12/1 -> Bus Creator1/12  "NegativeInsulationResistance"
  Data Type Conversion13/1 -> Bus Creator1/13  "PositiveInsulationResistance"
  Add/1 -> Data Store Write/1
  Data Store Read/1 -> Add/1
  Constant/1 -> Add/2

== system ZT_VehCtrl_18B_CAN/SigIn/CAN0 /BMS_Relay Status1/UNPACK ==
  ID : Inport
  data : Inport  Port=2
  length : Inport  Port=3
  timestamp : Inport  Port=4
  Action Port : ActionPort
  Bus Creator : BusCreator  Inputs=7  OutDataTypeStr=Bus: CAN_MESSAGE_BUS  NonVirtualBus=on
  Bus Creator1 : BusCreator  Inputs=17
  CAN Unpack6 : canmsglib/CAN Unpack  CANdbFile=D:\VCU\VCU_SL_ZhengZhou\ZT2\模型与接口\CAN_DBC\整车CANA_GBK.dbc  MsgList=(none)  MsgName=BMS_Relay_Status  MsgIDType=Standard (11-bit identifier)  MsgIdentifier=849  MsgLength=8  SignalInfo=Relay_ACChargeFaultStatus$16$2$2$2$1$0$1$0$0$3$#Relay_ACChargeStatus$4$1$2$2$1$0$1$0$0$1$#Relay_DCChargeFaultStatus$18$2$2$2$1$0$1$0$0$3$#Relay_DCChargeStatus$5$1$2$2$1$0$1$0$0$1$#Relay_DischargeFaultStatus$14$2$2$2$1$0$1$0$0$3$#Relay_DischargeStatus$3$1$2$2$1$0$1$0$0$1$#Relay_HeatingFaultStatus$20$2$2$2$1$0$1$0$0$3$#Relay_HeatingStatus$6$1$2$2$1$0$1$0$0$1$#Relay_NegativeFaultStatus$10$2$2$2$1$0$1$0$0$3$#Relay_NegativeStatus$1$1$2$2$1$0$1$0$0$1$#Relay_PositiveFaultStatus$8$2$2$2$1$0$1$0$0$1$#Relay_PositiveStatus$0$1$2$2$1$0$1$0$0$1$#Relay_PrechargeFaultStatus$12$2$2$2$1$0$1$0$0$3$#Relay_PrechargeStatus$2$1$2$2$1$0$1$0$0$1$#Relay_RefrigerationFaultStatus$22$2$2$2$1$0$1$0$0$3$#Relay_RefrigerationStatus$7$1$2$2$1$0$1$0$0$1$#  NSignals=16  IDPort=off  TimestampPort=off  ErrorPort=off  RemotePort=off  LengthPort=off  StatusPort=off  StartBits=str2num('[int32(16);int32(4);int32(18);int32(5);int32(14);int32(3);int32(20);int32(6);int32(10);int32(1);int32(8);int32(0);int32(12);int32(2);int32(22);int32(7)]')  SignalSizes=str2num('[int32(2);int32(1);int32(2);int32(1);int32(2);int32(1);int32(2);int32(1);int32(2);int32(1);int32(2);int32(1);int32(2);int32(1);int32(2);int32(1)]')  ByteOrders=str2num('[int32(2);int32(2);int32(2);int32(2);int32(2);int32(2);int32(2);int32(2);int32(2);int32(2);int32(2);int32(2);int32(2);int32(2);int32(2);int32(2)]')  DataTypes=str2num('[int32(2);int32(2);int32(2);int32(2);int32(2);int32(2);int32(2);int32(2);int32(2);int32(2);int32(2);int32(2);int32(2);int32(2);int32(2);int32(2)]')  MultiplexTypes=str2num('[int32(1);int32(1);int32(1);int32(1);int32(1);int32(1);int32(1);int32(1);int32(1);int32(1);int32(1);int32(1);int32(1);int32(1);int32(1);int32(1)]')  MultiplexValues=str2num('[double(0);double(0);double(0);double(0);double(0);double(0);double(0);double(0);double(0);double(0);double(0);double(0);double(0);double(0);double(0);double(0)]')  Factors=str2num('[double(1);double(1);double(1);double(1);double(1);double(1);double(1);double(1);double(1);double(1);double(1);double(1);double(1);double(1);double(1);double(1)]')  Offsets=str2num('[double(0);double(0);double(0);double(0);double(0);double(0);double(0);double(0);double(0);double(0);double(0);double(0);double(0);double(0);double(0);double(0)]')  Minimums=str2num('[double(0);double(0);double(0);double(0);double(0);double(0);double(0);double(0);double(0);double(0);double(0);double(0);double(0);double(0);double(0);double(0)]')  Maximums=str2num('[double(3);double(1);double(3);double(1);double(3);double(1);double(3);double(1);double(3);double(1);double(1);double(1);double(3);double(1);double(3);double(1)]')  ApplyMinMax=off
      settings: SourceProductName=Simulink Real-Time  SourceProductBaseCode=XP  DataFormat=CANdb specified signals
  Constant1 : Constant  Value=0  OutDataTypeStr=uint8
  Constant4 : Constant  Value=0  OutDataTypeStr=uint8
  Constant5 : Constant  Value=0  OutDataTypeStr=uint8
  Data Type Conversion{,14..15,17} (4 alike) : DataTypeConversion  OutDataTypeStr=uint8
  Data Type Conversion{1,4,6,8,10,12,16,21} (8 alike) : DataTypeConversion  OutDataTypeStr=boolean
  Data Type Conversion{2..3,5,7,9,11,13,20} (8 alike) : DataTypeConversion  OutDataTypeStr=single
  Data Type Conversion18 : DataTypeConversion  OutDataTypeStr=uint32
  Data Type Conversion19 : DataTypeConversion  OutDataTypeStr=double
  Message : Outport
  wires:
  Bus Creator1/1 -> Message/1
  Data Type Conversion15/1 -> Bus Creator/3  "Remote"
  Data Type Conversion14/1 -> Bus Creator/2  "Length"
  Data Type Conversion/1 -> Bus Creator/1  "Extended"
  Bus Creator/1 -> CAN Unpack6/1  "CAN_Msg_In"
  Data Type Conversion17/1 -> Bus Creator/4  "Error"
  timestamp/1 -> Data Type Conversion19/1
  Data Type Conversion19/1 -> Bus Creator/6  "Timestamp"
  ID/1 -> Data Type Conversion18/1
  Constant5/1 -> Data Type Conversion17/1
  Constant1/1 -> Data Type Conversion/1
  Data Type Conversion18/1 -> Bus Creator/5  "ID"
  data/1 -> Bus Creator/7  "Data"
  length/1 -> Data Type Conversion14/1
  Constant4/1 -> Data Type Conversion15/1
  CAN Unpack6/1 -> Data Type Conversion1/1
  CAN Unpack6/2 -> Data Type Conversion2/1
  CAN Unpack6/3 -> Data Type Conversion3/1
  CAN Unpack6/4 -> Data Type Conversion4/1
  CAN Unpack6/5 -> Data Type Conversion5/1
  CAN Unpack6/6 -> Data Type Conversion6/1
  CAN Unpack6/7 -> Data Type Conversion7/1
  CAN Unpack6/8 -> Data Type Conversion8/1
  CAN Unpack6/9 -> Data Type Conversion9/1
  CAN Unpack6/10 -> Data Type Conversion10/1
  CAN Unpack6/11 -> Data Type Conversion11/1
  CAN Unpack6/12 -> Data Type Conversion12/1
  CAN Unpack6/13 -> Data Type Conversion13/1
  CAN Unpack6/14 -> Data Type Conversion16/1
  CAN Unpack6/15 -> Data Type Conversion20/1
  CAN Unpack6/16 -> Data Type Conversion21/1
  Data Type Conversion1/1 -> Bus Creator1/1
  Data Type Conversion2/1 -> Bus Creator1/2  "Relay_ACChargeStatus"
  Data Type Conversion3/1 -> Bus Creator1/3
  Data Type Conversion4/1 -> Bus Creator1/4  "Relay_DCChargeStatus"
  Data Type Conversion5/1 -> Bus Creator1/5
  Data Type Conversion6/1 -> Bus Creator1/6  "Relay_DischargeStatus"
  Data Type Conversion7/1 -> Bus Creator1/7
  Data Type Conversion8/1 -> Bus Creator1/8  "Relay_HeatingStatus"
  Data Type Conversion9/1 -> Bus Creator1/9
  Data Type Conversion10/1 -> Bus Creator1/10  "Relay_NegativeStatus"
  Data Type Conversion11/1 -> Bus Creator1/11  "Relay_PositiveFaultStatus"
  Data Type Conversion12/1 -> Bus Creator1/12  "Relay_PositiveStatus"
  Data Type Conversion13/1 -> Bus Creator1/13
  Data Type Conversion16/1 -> Bus Creator1/14  "Relay_PrechargeStatus"
  Data Type Conversion20/1 -> Bus Creator1/15
  Data Type Conversion21/1 -> Bus Creator1/16  "Relay_RefrigerationStatus"
